simulink model "radia_hdiv_gpu_workflow"  (R2026a)
settings: Solver=FixedStepDiscrete  StopTime=.05  FixedStep=.01
model workspace (MAT data in the model file):
  hdivConfig.Backend = 'gpu'
  hdivConfig.Setup.schema = 'radia.hdiv-device-setup.v1'
  hdivConfig.Setup.backend = 'gpu'
  hdivConfig.Setup.family = 'hex'
  hdivConfig.Setup.mesh_sha256 = '8eb4f1f22fb78d2947513ee7af5941cbb44e4b25c591f9c315fce149b638d1f6'
  hdivConfig.Setup.label_contract_sha256 = '349426d9ef33d9cdfab82222c138b02cb9eb5f446d37baf75c8e66fe6de09df2'
  hdivConfig.Setup.order = 2
  hdivConfig.Setup.dofs = 207
  hdivConfig.Setup.rhs_operator = [0 0 0.5 0.5 0 -3.76786693363e-19 0 0.5 0.5 -2.8836279319e-35 -1.5741009319e-18 -4.51028103754e-17 ... (621 elements, 207x3)]
  hdivConfig.Setup.mean_operator = [0 8.91164892723e-20 0.25 0 -0.25 -8.91164892723e-20 0.25 0 0 0.25 0 0 ... (621 elements, 3x207)]
  hdivConfig.Setup.charges.cell_vertices = [0; 0; 0; 0.5; 0; 0; 1; 0; 0; 0; 0.5; 0; 0.5; 0.5; 0; 1; 0.5; 0; 0; 1; 0; 0.5; 1; 0; 1; 1; 0; 0; 0; 0.5; 0.5; 0; 0.5; 1; 0; 0.5; 0; 0.5; 0.5; 0.5; 0.5; 0.5; 1; 0.5; 0.5; 0; 1; 0.5; 0.5; 1; 0.5; 1; 1; 0.5; 0; 0; 1; 0.5; 0; 1; 1; 0; 1; 0; 0.5; 1; 0.5; 0.5; 1; 1; 0.5; 1; 0; 1; 1; 0.5; 1; 1; 1; 1; 1; 0; 0; 1; 0.5; 0; 1; 1; 0; 1; 0; 0.5; 1; 0.5; 0.5; 1; 1; 0.5; 1; 0; 1; 1; 0.5; 1; 1; 1; 1; 1; 0; 0; 1.5; 0.5; 0; 1.5; 1; 0; 1.5; 0; 0.5; 1.5; 0.5; 0.5; 1.5; 1; 0.5; 1.5; 0; 1; 1.5; 0.5; 1; 1.5; 1; 1; 1.5; 0; 0; 2; 0.5; 0; 2; 1; 0; 2; 0; 0.5; 2; 0.5; 0.5; 2; 1; 0.5; 2; 0; 1; 2; 0.5; 1; 2; 1; 1; 2]
  hdivConfig.Setup.charges.face_vertices = [0; 0; 0; 0; 0.5; 0; 0; 1; 0; 0.5; 0; 0; 0.5; 0.5; 0; 0.5; 1; 0; 1; 0; 0; 1; 0.5; 0; 1; 1; 0; 0; 0; 0; 0.5; 0; 0; 1; 0; 0; 0; 0; 0.5; 0.5; 0; 0.5; 1; 0; 0.5; 0; 0; 1; 0.5; 0; 1; 1; 0; 1; 1; 0; 0; 1; 0.5; 0; 1; 1; 0; 1; 0; 0.5; 1; 0.5; 0.5; 1; 1; 0.5; 1; 0; 1; 1; 0.5; 1; 1; 1; 1; 1; 1; 0; 0.5; 1; 0; 0; 1; 0; 1; 1; 0.5; 0.5; 1; 0.5; 0; 1; 0.5; 1; 1; 1; 0.5; 1; 1; 0; 1; 1; 0; 1; 0; 0; 0.5; 0; 0; 0; 0; 0; 1; 0.5; 0; 0.5; 0.5; 0; 0; 0.5; 0; 1; 1; 0; 0.5; 1; 0; 0; 1; 0; 0; 2; 0.5; 0; 2; 1; 0; 2; 0; 0.5; 2; 0.5; 0.5; 2; 1; 0.5; 2; 0; 1; 2; 0.5; 1; 2; 1; 1; 2; 0; 0; 1; 0.5; 0; 1; 1; 0; 1; 0; 0; 1.5; 0.5; 0; 1.5; 1; 0; 1.5; 0; 0; 2; 0.5; 0; 2; 1; 0; 2; 1; 0; 1; 1; 0.5; 1; 1; 1; 1; 1; 0; 1.5; 1; 0.5; 1.5; 1; 1; 1.5; 1; 0; 2; 1; 0.5; 2; 1; 1; 2; 1; 1; 1; 0.5; 1; 1; 0; 1; 1; 1; 1; 1.5; 0.5; 1; 1.5; 0; 1; 1.5; 1; 1; 2; 0.5; 1; 2; 0; 1; 2; 0; 1; 1; 0; 0.5; 1; 0; 0; 1; 0; 1; 1.5; 0; 0.5; 1.5; 0; 0; 1.5; 0; 1; 2; 0; 0.5; 2; 0; 0; 2]
  hdivConfig.Setup.charges.tet_rule = []
  hdivConfig.Setup.charges.tri_rule = []
  hdivConfig.Setup.charges.tet_low_rule = []
  hdivConfig.Setup.charges.tri_low_rule = []
  hdivConfig.Setup.charges.cell_tables = [1 -1 -1 -1 -1 1 0 0 0 0 0 0 ... (2916 elements, 2916x1)]
  hdivConfig.Setup.charges.face_tables = [-1 8 8 7.99999999999 7.99999999998 -4 -4 4 4 -1.86850535044e-13 -16 -48 ... (324 elements, 324x1)]
  hdivConfig.Setup.charges.charge_host = [0; 0; 0; 0; 0; 0; 0; 0; 0; 0; 0; 0; 0; 0; 0; 0; 0; 0; 0; 0; 0; 0; 0; 0; 0; 0; 0; 1; 1; 1; 1; 1; 1; 1; 1; 1; 1; 1; 1; 1; 1; 1; 1; 1; 1; 1; 1; 1; 1; 1; 1; 1; 1; 1; 0; 0; 0; 0; 0; 0; 0; 0; 0; 1; 1; 1; 1; 1; 1; 1; 1; 1; 2; 2; 2; 2; 2; 2; 2; 2; 2; 3; 3; 3; 3; 3; 3; 3; 3; 3; 4; 4; 4; 4; 4; 4; 4; 4; 4; 5; 5; 5; 5; 5; 5; 5; 5; 5; 6; 6; 6; 6; 6; 6; 6; 6; 6; 7; 7; 7; 7; 7; 7; 7; 7; 7; 8; 8; 8; 8; 8; 8; 8; 8; 8; 9; 9; 9; 9; 9; 9; 9; 9; 9]
  hdivConfig.Setup.charges.charge_kind = [0; 0; 0; 0; 0; 0; 0; 0; 0; 0; 0; 0; 0; 0; 0; 0; 0; 0; 0; 0; 0; 0; 0; 0; 0; 0; 0; 0; 0; 0; 0; 0; 0; 0; 0; 0; 0; 0; 0; 0; 0; 0; 0; 0; 0; 0; 0; 0; 0; 0; 0; 0; 0; 0; 1; 1; 1; 1; 1; 1; 1; 1; 1; 1; 1; 1; 1; 1; 1; 1; 1; 1; 1; 1; 1; 1; 1; 1; 1; 1; 1; 1; 1; 1; 1; 1; 1; 1; 1; 1; 1; 1; 1; 1; 1; 1; 1; 1; 1; 1; 1; 1; 1; 1; 1; 1; 1; 1; 1; 1; 1; 1; 1; 1; 1; 1; 1; 1; 1; 1; 1; 1; 1; 1; 1; 1; 1; 1; 1; 1; 1; 1; 1; 1; 1; 1; 1; 1; 1; 1; 1; 1; 1; 1]
  hdivConfig.Setup.charges.charge_exponents = [0; 0; 0; 1; 0; 0; 2; 0; 0; 0; 1; 0; 1; 1; 0; 2; 1; 0; 0; 2; 0; 1; 2; 0; 2; 2; 0; 0; 0; 1; 1; 0; 1; 2; 0; 1; 0; 1; 1; 1; 1; 1; 2; 1; 1; 0; 2; 1; 1; 2; 1; 2; 2; 1; 0; 0; 2; 1; 0; 2; 2; 0; 2; 0; 1; 2; 1; 1; 2; 2; 1; 2; 0; 2; 2; 1; 2; 2; 2; 2; 2; 0; 0; 0; 1; 0; 0; 2; 0; 0; 0; 1; 0; 1; 1; 0; 2; 1; 0; 0; 2; 0; 1; 2; 0; 2; 2; 0; 0; 0; 1; 1; 0; 1; 2; 0; 1; 0; 1; 1; 1; 1; 1; 2; 1; 1; 0; 2; 1; 1; 2; 1; 2; 2; 1; 0; 0; 2; 1; 0; 2; 2; 0; 2; 0; 1; 2; 1; 1; 2; 2; 1; 2; 0; 2; 2; 1; 2; 2; 2; 2; 2; 0; 0; 0; 1; 0; 0; 2; 0; 0; 0; 1; 0; 1; 1; 0; 2; 1; 0; 0; 2; 0; 1; 2; 0; 2; 2; 0; 0; 0; 0; 1; 0; 0; 2; 0; 0; 0; 1; 0; 1; 1; 0; 2; 1; 0; 0; 2; 0; 1; 2; 0; 2; 2; 0; 0; 0; 0; 1; 0; 0; 2; 0; 0; 0; 1; 0; 1; 1; 0; 2; 1; 0; 0; 2; 0; 1; 2; 0; 2; 2; 0; 0; 0; 0; 1; 0; 0; 2; 0; 0; 0; 1; 0; 1; 1; 0; 2; 1; 0; 0; 2; 0; 1; 2; 0; 2; 2; 0; 0; 0; 0; 1; 0; 0; 2; 0; 0; 0; 1; 0; 1; 1; 0; 2; 1; 0; 0; 2; 0; 1; 2; 0; 2; 2; 0; 0; 0; 0; 1; 0; 0; 2; 0; 0; 0; 1; 0; 1; 1; 0; 2; 1; 0; 0; 2; 0; 1; 2; 0; 2; 2; 0; 0; 0; 0; 1; 0; 0; 2; 0; 0; 0; 1; 0; 1; 1; 0; 2; 1; 0; 0; 2; 0; 1; 2; 0; 2; 2; 0; 0; 0; 0; 1; 0; 0; 2; 0; 0; 0; 1; 0; 1; 1; 0; 2; 1; 0; 0; 2; 0; 1; 2; 0; 2; 2; 0; 0; 0; 0; 1; 0; 0; 2; 0; 0; 0; 1; 0; 1; 1; 0; 2; 1; 0; 0; 2; 0; 1; 2; 0; 2; 2; 0; 0; 0; 0; 1; 0; 0; 2; 0; 0; 0; 1; 0; 1; 1; 0; 2; 1; 0; 0; 2; 0; 1; 2; 0; 2; 2; 0]
  hdivConfig.Setup.charges.cell_class = [0; 0]
  hdivConfig.Setup.charges.cell_dofs = [0; 5; 1; 3; 4; 2; 11; 12; 13; 14; 15; 16; 17; 18; 51; 52; 53; 54; 55; 56; 57; 58; 19; 20; 21; 22; 23; 24; 25; 26; 35; 36; 37; 38; 39; 40; 41; 42; 43; 44; 45; 46; 47; 48; 49; 50; 27; 28; 29; 30; 31; 32; 33; 34; 99; 100; 101; 102; 103; 104; 105; 106; 107; 108; 109; 110; 111; 112; 113; 114; 115; 116; 117; 118; 119; 120; 121; 122; 123; 124; 125; 126; 127; 128; 129; 130; 131; 132; 133; 134; 135; 136; 137; 138; 139; 140; 141; 142; 143; 144; 145; 146; 147; 148; 149; 150; 151; 152; 5; 10; 6; 8; 9; 7; 51; 52; 53; 54; 55; 56; 57; 58; 91; 92; 93; 94; 95; 96; 97; 98; 59; 60; 61; 62; 63; 64; 65; 66; 75; 76; 77; 78; 79; 80; 81; 82; 83; 84; 85; 86; 87; 88; 89; 90; 67; 68; 69; 70; 71; 72; 73; 74; 153; 154; 155; 156; 157; 158; 159; 160; 161; 162; 163; 164; 165; 166; 167; 168; 169; 170; 171; 172; 173; 174; 175; 176; 177; 178; 179; 180; 181; 182; 183; 184; 185; 186; 187; 188; 189; 190; 191; 192; 193; 194; 195; 196; 197; 198; 199; 200; 201; 202; 203; 204; 205; 206]
  hdivConfig.Setup.charges.cell_exponents = [0; 0; 0; 1; 0; 0; 2; 0; 0; 0; 1; 0; 1; 1; 0; 2; 1; 0; 0; 2; 0; 1; 2; 0; 2; 2; 0; 0; 0; 1; 1; 0; 1; 2; 0; 1; 0; 1; 1; 1; 1; 1; 2; 1; 1; 0; 2; 1; 1; 2; 1; 2; 2; 1; 0; 0; 2; 1; 0; 2; 2; 0; 2; 0; 1; 2; 1; 1; 2; 2; 1; 2; 0; 2; 2; 1; 2; 2; 2; 2; 2]
  hdivConfig.Setup.charges.face_class = [0; 1; 1; 1; 2; 3; 1; 1; 1; 2]
  hdivConfig.Setup.charges.face_dofs = [0; 11; 12; 13; 14; 15; 16; 17; 18; 1; 19; 20; 21; 22; 23; 24; 25; 26; 3; 35; 36; 37; 38; 39; 40; 41; 42; 4; 43; 44; 45; 46; 47; 48; 49; 50; 2; 27; 28; 29; 30; 31; 32; 33; 34; 10; 91; 92; 93; 94; 95; 96; 97; 98; 6; 59; 60; 61; 62; 63; 64; 65; 66; 8; 75; 76; 77; 78; 79; 80; 81; 82; 9; 83; 84; 85; 86; 87; 88; 89; 90; 7; 67; 68; 69; 70; 71; 72; 73; 74]
  hdivConfig.Setup.charges.face_exponents = [0; 0; 1; 0; 2; 0; 0; 1; 1; 1; 2; 1; 0; 2; 1; 2; 2; 2]
  hdivConfig.Setup.charges.hex_rules = [0; 0.0469100770307; 0.118463442528; 0; 0.230765344947; 0.23931433525; 0; 0.5; 0.284444444444; 0; 0.769234655053; 0.23931433525; 0; 0.953089922969; 0.118463442528; 1; 0.0254460438286; 0.0647424830844; 1; 0.1292344072; 0.139852695745; 1; 0.297077424311; 0.190915025253; 1; 0.5; 0.208979591837; 1; 0.702922575689; 0.190915025253; 1; 0.8707655928; 0.139852695745; 1; 0.974553956171; 0.0647424830844; 2; 0.0337652428984; 0.0856622461896; 2; 0.169395306767; 0.180380786524; 2; 0.380690406958; 0.233956967286; 2; 0.619309593042; 0.233956967286; 2; 0.830604693233; 0.180380786524; 2; 0.966234757102; 0.0856622461896; 3; 0.0337652428984; 0.0856622461896; 3; 0.169395306767; 0.180380786524; 3; 0.380690406958; 0.233956967286; 3; 0.619309593042; 0.233956967286; 3; 0.830604693233; 0.180380786524; 3; 0.966234757102; 0.0856622461896]
  hdivConfig.Setup.charges.hex_bands = [1; 1]
  hdivConfig.Setup.charges.family = 'hex'
  hdivConfig.Setup.charges.far_factor = 1e+30
  hdivConfig.Setup.charges.compression = 'aca'
  hdivConfig.Setup.charges.dofs = 207
  hdivConfig.Setup.charges.aca.eps = 1e-10
  hdivConfig.Setup.charges.aca.eta = 2
  hdivConfig.Setup.charges.aca.leaf_size = 64
  hdivConfig.Setup.charges.aca.max_rank = 200
  hdivConfig.Setup.charges.aca.rank_cap = 'dense'
  hdivConfig.Setup.evaluation.rule = [0.0254460438286 0.0254460438286 0.0254460438286 0.000271373887435 0.0254460438286 0.0254460438286 0.1292344072 0.000586205037318 0.0254460438286 0.0254460438286 0.297077424311 0.000800237341918 ... (1372 elements, 1372x1)]
  hdivConfig.Setup.evaluation.reference_shapes = [0 0 0.974553956171 0 0 0.0254460438286 0 -0.974553956171 0 0.0254460438286 0 0 ... (111132 elements, 111132x1)]
  hdivConfig.Setup.evaluation.vertices = [0; 0; 0; 0.5; 0; 0; 1; 0; 0; 0; 0.5; 0; 0.5; 0.5; 0; 1; 0.5; 0; 0; 1; 0; 0.5; 1; 0; 1; 1; 0; 0; 0; 0.5; 0.5; 0; 0.5; 1; 0; 0.5; 0; 0.5; 0.5; 0.5; 0.5; 0.5; 1; 0.5; 0.5; 0; 1; 0.5; 0.5; 1; 0.5; 1; 1; 0.5; 0; 0; 1; 0.5; 0; 1; 1; 0; 1; 0; 0.5; 1; 0.5; 0.5; 1; 1; 0.5; 1; 0; 1; 1; 0.5; 1; 1; 1; 1; 1; 0; 0; 1; 0.5; 0; 1; 1; 0; 1; 0; 0.5; 1; 0.5; 0.5; 1; 1; 0.5; 1; 0; 1; 1; 0.5; 1; 1; 1; 1; 1; 0; 0; 1.5; 0.5; 0; 1.5; 1; 0; 1.5; 0; 0.5; 1.5; 0.5; 0.5; 1.5; 1; 0.5; 1.5; 0; 1; 1.5; 0.5; 1; 1.5; 1; 1; 1.5; 0; 0; 2; 0.5; 0; 2; 1; 0; 2; 0; 0.5; 2; 0.5; 0.5; 2; 1; 0.5; 2; 0; 1; 2; 0.5; 1; 2; 1; 1; 2]
  hdivConfig.Setup.evaluation.element_class = [0; 0]
  hdivConfig.Setup.evaluation.element_dofs = [0; 5; 1; 3; 4; 2; 11; 12; 13; 14; 15; 16; 17; 18; 51; 52; 53; 54; 55; 56; 57; 58; 19; 20; 21; 22; 23; 24; 25; 26; 35; 36; 37; 38; 39; 40; 41; 42; 43; 44; 45; 46; 47; 48; 49; 50; 27; 28; 29; 30; 31; 32; 33; 34; 99; 100; 101; 102; 103; 104; 105; 106; 107; 108; 109; 110; 111; 112; 113; 114; 115; 116; 117; 118; 119; 120; 121; 122; 123; 124; 125; 126; 127; 128; 129; 130; 131; 132; 133; 134; 135; 136; 137; 138; 139; 140; 141; 142; 143; 144; 145; 146; 147; 148; 149; 150; 151; 152; 5; 10; 6; 8; 9; 7; 51; 52; 53; 54; 55; 56; 57; 58; 91; 92; 93; 94; 95; 96; 97; 98; 59; 60; 61; 62; 63; 64; 65; 66; 75; 76; 77; 78; 79; 80; 81; 82; 83; 84; 85; 86; 87; 88; 89; 90; 67; 68; 69; 70; 71; 72; 73; 74; 153; 154; 155; 156; 157; 158; 159; 160; 161; 162; 163; 164; 165; 166; 167; 168; 169; 170; 171; 172; 173; 174; 175; 176; 177; 178; 179; 180; 181; 182; 183; 184; 185; 186; 187; 188; 189; 190; 191; 192; 193; 194; 195; 196; 197; 198; 199; 200; 201; 202; 203; 204; 205; 206]
  hdivConfig.Setup.evaluation.element_points = [0 1 2 3 4 5 6 7 8 9 10 11 ... (686 elements, 686x1)]
  hdivConfig.AppliedField = [1000 -2000 5000]
  hdivConfig.BHTable = [0  0; 10  0.0125785181227; 100  0.125372159591; 500  0.581341865069; 2000  1.21394605949; 10000  1.26920342687]
  hdivConfig.NumDoF = 207
  hdivConfig.Preconditioner = 'reference-diagonal'
  hdivConfig.SampleTime = 0.01
  hdivConfig.RunDirectory = 'radia_hdiv_gpu_runs'
  triggerSignal.time = [0; 0.01; 0.02; 0.03; 0.04; 0.05]
  triggerSignal.signals.values = [0; 1; 1; 0; 1; 0]
  triggerSignal.signals.dimensions = 1
settings Model: ModifiedByFormat=Radia Development Team  Creator=Radia Development Team  LastModifiedBy=Radia Development Team

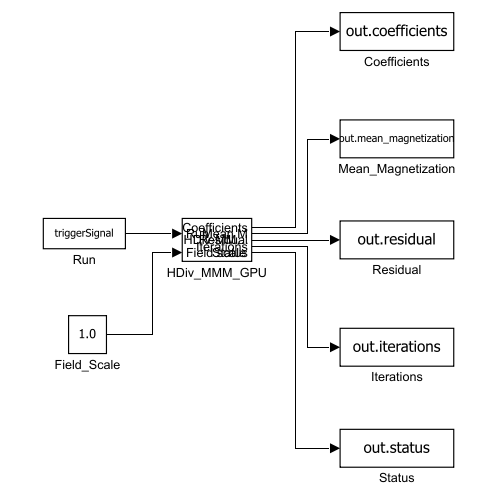
[thumbnail: Simulink's stored preview of the top-level diagram]
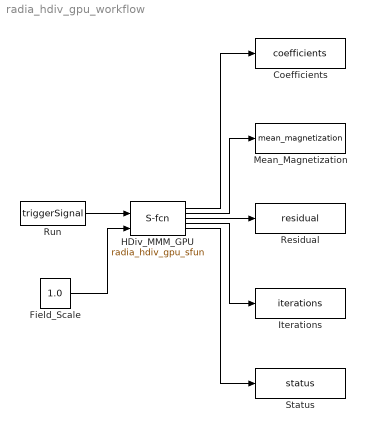
== system radia_hdiv_gpu_workflow ==
  Coefficients : ToWorkspace  VariableName=coefficients  SaveFormat=Structure With Time  SampleTime=-1
  Field_Scale : Constant  Value=1.0
  HDiv_MMM_GPU : M-S-Function  FunctionName=radia_hdiv_gpu_sfun  Parameters=hdivConfig  mask(Radia Shared HDiv GPU Workflow){}
      mask help: Explicit rising trigger; shared CUDA BH/Newton. Held outputs update on the next sample. No coil circuit model or CPU fallback.
      mask Display: disp('HDiv-MMM GPU'); port_label('input',1,'Run'); port_label('input',2,'Field scale'); port_label('output',1,'Coefficients'); port_label('output',2,'Mean M'); port_label('output',3,'Residual'); port_label('output',4,'Iterations'); port_label('output',5,'Status');
  Iterations : ToWorkspace  VariableName=iterations  SaveFormat=Structure With Time  SampleTime=-1
  Mean_Magnetization : ToWorkspace  VariableName=mean_magnetization  SaveFormat=Structure With Time  SampleTime=-1
  Residual : ToWorkspace  VariableName=residual  SaveFormat=Structure With Time  SampleTime=-1
  Run : FromWorkspace  VariableName=triggerSignal  SampleTime=.01  Interpolate=off  OutputAfterFinalValue=Holding final value
  Status : ToWorkspace  VariableName=status  SaveFormat=Structure With Time  SampleTime=-1
  wires:
  HDiv_MMM_GPU/5 -> Status/1
  HDiv_MMM_GPU/4 -> Iterations/1
  HDiv_MMM_GPU/3 -> Residual/1
  HDiv_MMM_GPU/2 -> Mean_Magnetization/1
  Field_Scale/1 -> HDiv_MMM_GPU/2
  HDiv_MMM_GPU/1 -> Coefficients/1
  Run/1 -> HDiv_MMM_GPU/1
